simulink model "Benchmark_model"  (R2018a)
settings: Solver=ode1  StartTime=0  StopTime=t_end  FixedStep=simTs  RelTol=1e-3  EnableMultiTasking=on
values from neighbouring files (symbols this model uses):
  driv_rect_time = 0.5    [Initial_parameters.m]
  gamma = 25    [Initial_parameters.m]
  hw_min = 3    [Initial_parameters.m]
  Initial_eng_spd = 0    [Initial_parameters.m]
  Initial_headway = Sensor_FOL_dDist(2)    [Initial_parameters.m]
  Initial_SOC = 50    [Initial_parameters.m]
  Initial_vhcl_spd = 0    [Initial_parameters.m]
  spd_lim = 60    [Initial_parameters.m]
undefined symbols (not defined in the file or in its folder): Route_Distance, Route_Slope
(part 2 of 2)

== matlab function Benchmark_model/Traffic Scenario/V2I information/Data arrangement ==
  data: ego_distance input; State_next1 output; tRemain_next1 output; s2inters_next1 output; State_next2 output; tRemain_next2 output; state_sum input; tRemain_sum input; s2inters_next2 output
function [State_next1,tRemain_next1,s2inters_next1,State_next2,tRemain_next2,s2inters_next2] = fcn(ego_distance,state_sum,tRemain_sum)

%%%% state
TrfLight_TL1_State = state_sum(1);
TrfLight_TL2_State = state_sum(2);
TrfLight_TL3_State = state_sum(3);
TrfLight_TL4_State = state_sum(4);
TrfLight_TL5_State = state_sum(5);
TrfLight_TL6_State = state_sum(6);
TrfLight_TL7_State = state_sum(7);
TrfLight_TL8_State = state_sum(8);
TrfLight_TL9_State = state_sum(9);
TrfLight_TL10_State = state_sum(10);
TrfLight_TL11_State = state_sum(11);
TrfLight_TL12_State = state_sum(12);
TrfLight_TL13_State = state_sum(13);
TrfLight_TL14_State = state_sum(14);
TrfLight_TL15_State = state_sum(15);
TrfLight_TL16_State = state_sum(16);
TrfLight_TL17_State = state_sum(17);
TrfLight_TL18_State = state_sum(18);
TrfLight_TL19_State = state_sum(19);
TrfLight_TL20_State = state_sum(20);
TrfLight_TL21_State = state_sum(21);
TrfLight_TL22_State = state_sum(22);
TrfLight_TL23_State = state_sum(23);
TrfLight_TL24_State = state_sum(24);
TrfLight_TL25_State = state_sum(25);
TrfLight_TL26_State = state_sum(26);

%%%% tRemain
TrfLight_TL1_tRemain = tRemain_sum(1);
TrfLight_TL2_tRemain = tRemain_sum(2);
TrfLight_TL3_tRemain = tRemain_sum(3);
TrfLight_TL4_tRemain = tRemain_sum(4);
TrfLight_TL5_tRemain = tRemain_sum(5);
TrfLight_TL6_tRemain = tRemain_sum(6);
TrfLight_TL7_tRemain = tRemain_sum(7);
TrfLight_TL8_tRemain = tRemain_sum(8);
TrfLight_TL9_tRemain = tRemain_sum(9);
TrfLight_TL10_tRemain = tRemain_sum(10);
TrfLight_TL11_tRemain = tRemain_sum(11);
TrfLight_TL12_tRemain = tRemain_sum(12);
TrfLight_TL13_tRemain = tRemain_sum(13);
TrfLight_TL14_tRemain = tRemain_sum(14);
TrfLight_TL15_tRemain = tRemain_sum(15);
TrfLight_TL16_tRemain = tRemain_sum(16);
TrfLight_TL17_tRemain = tRemain_sum(17);
TrfLight_TL18_tRemain = tRemain_sum(18);
TrfLight_TL19_tRemain = tRemain_sum(19);
TrfLight_TL20_tRemain = tRemain_sum(20);
TrfLight_TL21_tRemain = tRemain_sum(21);
TrfLight_TL22_tRemain = tRemain_sum(22);
TrfLight_TL23_tRemain = tRemain_sum(23);
TrfLight_TL24_tRemain = tRemain_sum(24);
TrfLight_TL25_tRemain = tRemain_sum(25);
TrfLight_TL26_tRemain = tRemain_sum(26);

intersection = [1288;
2358;
2572;
2886;
3066;
3150;
3422;
3784;
4696;
5377;
5576;
6855;
7626;
10162;
10575;
10948;
11201;
11537;
11781;
12302;
12587;
12785;
13032;
13368;
14364;
15082]; % original position of the intersection to the departure


intersection = intersection-3.2; 
% the vehicle length should be considered at the departure 
% and at the departure, the distance of ego vehicle to the first intesection is actually 1284.8 [m]
% so a correction of 3.2 [m] is given.

distination = 16002;


           
if ego_distance < intersection(1)
    TrfLight_State_sum_next1 = TrfLight_TL1_State;
    TrfLight_tRemain_sum_next1 = TrfLight_TL1_tRemain;
    TrfLight_State_sum_next2 = TrfLight_TL2_State;
    TrfLight_tRemain_sum_next2 = TrfLight_TL2_tRemain;  
    ego_vehicle_s2_inters_next1 = intersection(1)-ego_distance;
    ego_vehicle_s2_inters_next2 = intersection(2)-ego_distance;
elseif ego_distance < intersection(2)
    TrfLight_State_sum_next1 = TrfLight_TL2_State;
    TrfLight_tRemain_sum_next1 = TrfLight_TL2_tRemain; 
    TrfLight_State_sum_next2 = TrfLight_TL3_State;
    TrfLight_tRemain_sum_next2 = TrfLight_TL3_tRemain;
    ego_vehicle_s2_inters_next1 = intersection(2)-ego_distance;
    ego_vehicle_s2_inters_next2 = intersection(3)-ego_distance;
elseif ego_distance < intersection(3)
    TrfLight_State_sum_next1 = TrfLight_TL3_State;
    TrfLight_tRemain_sum_next1 = TrfLight_TL3_tRemain; 
    TrfLight_State_sum_next2 = TrfLight_TL4_State;
    TrfLight_tRemain_sum_next2 = TrfLight_TL4_tRemain; 
    ego_vehicle_s2_inters_next1 = intersection(3)-ego_distance;
    ego_vehicle_s2_inters_next2 = intersection(4)-ego_distance;
elseif ego_distance < intersection(4)
    TrfLight_State_sum_next1 = TrfLight_TL4_State;
    TrfLight_tRemain_sum_next1 = TrfLight_TL4_tRemain; 
    TrfLight_State_sum_next2 = TrfLight_TL5_State;
    TrfLight_tRemain_sum_next2 = TrfLight_TL5_tRemain; 
    ego_vehicle_s2_inters_next1 = intersection(4)-ego_distance;
    ego_vehicle_s2_inters_next2 = intersection(5)-ego_distance;
elseif ego_distance < intersection(5)
    TrfLight_State_sum_next1 = TrfLight_TL5_State;
    TrfLight_tRemain_sum_next1 = TrfLight_TL5_tRemain;
    TrfLight_State_sum_next2 = TrfLight_TL6_State;
    TrfLight_tRemain_sum_next2 = TrfLight_TL6_tRemain;
    ego_vehicle_s2_inters_next1 = intersection(5)-ego_distance;
    ego_vehicle_s2_inters_next2 = intersection(6)-ego_distance;
elseif ego_distance < intersection(6)
    TrfLight_State_sum_next1 = TrfLight_TL6_State;
    TrfLight_tRemain_sum_next1 = TrfLight_TL6_tRemain;
    TrfLight_State_sum_next2 = TrfLight_TL7_State;
    TrfLight_tRemain_sum_next2 = TrfLight_TL7_tRemain;
    ego_vehicle_s2_inters_next1 = intersection(6)-ego_distance;
    ego_vehicle_s2_inters_next2 = intersection(7)-ego_distance;
elseif ego_distance < intersection(7)
    TrfLight_State_sum_next1 = TrfLight_TL7_State;
    TrfLight_tRemain_sum_next1 = TrfLight_TL7_tRemain;
    TrfLight_State_sum_next2 = TrfLight_TL8_State;
    TrfLight_tRemain_sum_next2 = TrfLight_TL8_tRemain; 
    ego_vehicle_s2_inters_next1 = intersection(7)-ego_distance;
    ego_vehicle_s2_inters_next2 = intersection(8)-ego_distance;
elseif ego_distance < intersection(8)
    TrfLight_State_sum_next1 = TrfLight_TL8_State;
    TrfLight_tRemain_sum_next1 = TrfLight_TL8_tRemain; 
    TrfLight_State_sum_next2 = TrfLight_TL9_State;
    TrfLight_tRemain_sum_next2 = TrfLight_TL9_tRemain;
    ego_vehicle_s2_inters_next1 = intersection(8)-ego_distance;
    ego_vehicle_s2_inters_next2 = intersection(9)-ego_distance;
elseif ego_distance < intersection(9)
    TrfLight_State_sum_next1 = TrfLight_TL9_State;
    TrfLight_tRemain_sum_next1 = TrfLight_TL9_tRemain; 
    TrfLight_State_sum_next2 = TrfLight_TL10_State;
    TrfLight_tRemain_sum_next2 = TrfLight_TL10_tRemain; 
    ego_vehicle_s2_inters_next1 = intersection(9)-ego_distance;
    ego_vehicle_s2_inters_next2 = intersection(10)-ego_distance;
elseif ego_distance < intersection(10)
    TrfLight_State_sum_next1 = TrfLight_TL10_State;
    TrfLight_tRemain_sum_next1 = TrfLight_TL10_tRemain;
    TrfLight_State_sum_next2 = TrfLight_TL11_State;
    TrfLight_tRemain_sum_next2 = TrfLight_TL11_tRemain; 
    ego_vehicle_s2_inters_next1 = intersection(10)-ego_distance;
    ego_vehicle_s2_inters_next2 = intersection(11)-ego_distance;
elseif ego_distance < intersection(11)
    TrfLight_State_sum_next1 = TrfLight_TL11_State;
    TrfLight_tRemain_sum_next1 = TrfLight_TL11_tRemain; 
    TrfLight_State_sum_next2 = TrfLight_TL12_State;
    TrfLight_tRemain_sum_next2 = TrfLight_TL12_tRemain; 
    ego_vehicle_s2_inters_next1 = intersection(11)-ego_distance;
    ego_vehicle_s2_inters_next2 = intersection(12)-ego_distance;
elseif ego_distance < intersection(12)
    TrfLight_State_sum_next1 = TrfLight_TL12_State;
    TrfLight_tRemain_sum_next1 = TrfLight_TL12_tRemain;
    TrfLight_State_sum_next2 = TrfLight_TL13_State;
    TrfLight_tRemain_sum_next2 = TrfLight_TL13_tRemain;
    ego_vehicle_s2_inters_next1 = intersection(12)-ego_distance;
    ego_vehicle_s2_inters_next2 = intersection(13)-ego_distance;
elseif ego_distance < intersection(13)
    TrfLight_State_sum_next1 = TrfLight_TL13_State;
    TrfLight_tRemain_sum_next1 = TrfLight_TL13_tRemain;
    TrfLight_State_sum_next2 = TrfLight_TL14_State;
    TrfLight_tRemain_sum_next2 = TrfLight_TL14_tRemain;
    ego_vehicle_s2_inters_next1 = intersection(13)-ego_distance;
    ego_vehicle_s2_inters_next2 = intersection(14)-ego_distance;
elseif ego_distance < intersection(14)
    TrfLight_State_sum_next1 = TrfLight_TL14_State;
    TrfLight_tRemain_sum_next1 = TrfLight_TL14_tRemain; 
    TrfLight_State_sum_next2 = TrfLight_TL15_State;
    TrfLight_tRemain_sum_next2 = TrfLight_TL15_tRemain;
    ego_vehicle_s2_inters_next1 = intersection(14)-ego_distance;
    ego_vehicle_s2_inters_next2 = intersection(15)-ego_distance;
elseif ego_distance < intersection(15)
    TrfLight_State_sum_next1 = TrfLight_TL15_State;
    TrfLight_tRemain_sum_next1 = TrfLight_TL15_tRemain; 
    TrfLight_State_sum_next2 = TrfLight_TL16_State;
    TrfLight_tRemain_sum_next2 = TrfLight_TL16_tRemain; 
    ego_vehicle_s2_inters_next1 = intersection(15)-ego_distance;
    ego_vehicle_s2_inters_next2 = intersection(16)-ego_distance;
elseif ego_distance < intersection(16)
    TrfLight_State_sum_next1 = TrfLight_TL16_State;
    TrfLight_tRemain_sum_next1 = TrfLight_TL16_tRemain; 
    TrfLight_State_sum_next2 = TrfLight_TL17_State;
    TrfLight_tRemain_sum_next2 = TrfLight_TL17_tRemain;
    ego_vehicle_s2_inters_next1 = intersection(16)-ego_distance;
    ego_vehicle_s2_inters_next2 = intersection(17)-ego_distance;
elseif ego_distance < intersection(17)
    TrfLight_State_sum_next1 = TrfLight_TL17_State;
    TrfLight_tRemain_sum_next1 = TrfLight_TL17_tRemain; 
    TrfLight_State_sum_next2 = TrfLight_TL18_State;
    TrfLight_tRemain_sum_next2 = TrfLight_TL18_tRemain;
    ego_vehicle_s2_inters_next1 = intersection(17)-ego_distance;
    ego_vehicle_s2_inters_next2 = intersection(18)-ego_distance;
elseif ego_distance < intersection(18)
    TrfLight_State_sum_next1 = TrfLight_TL18_State;
    TrfLight_tRemain_sum_next1 = TrfLight_TL18_tRemain; 
    TrfLight_State_sum_next2 = TrfLight_TL19_State;
    TrfLight_tRemain_sum_next2 = TrfLight_TL19_tRemain;
    ego_vehicle_s2_inters_next1 = intersection(18)-ego_distance;
    ego_vehicle_s2_inters_next2 = intersection(19)-ego_distance;
elseif ego_distance < intersection(19)
    TrfLight_State_sum_next1 = TrfLight_TL19_State;
    TrfLight_tRemain_sum_next1 = TrfLight_TL19_tRemain; 
    TrfLight_State_sum_next2 = TrfLight_TL20_State;
    TrfLight_tRemain_sum_next2 = TrfLight_TL20_tRemain; 
    ego_vehicle_s2_inters_next1 = intersection(19)-ego_distance;
    ego_vehicle_s2_inters_next2 = intersection(20)-ego_distance;
elseif ego_distance < intersection(20)
    TrfLight_State_sum_next1 = TrfLight_TL20_State;
    TrfLight_tRemain_sum_next1 = TrfLight_TL20_tRemain; 
    TrfLight_State_sum_next2 = TrfLight_TL21_State;
    TrfLight_tRemain_sum_next2 = TrfLight_TL21_tRemain; 
    ego_vehicle_s2_inters_next1 = intersection(20)-ego_distance;
    ego_vehicle_s2_inters_next2 = intersection(21)-ego_distance;
elseif ego_distance < intersection(21)
    TrfLight_State_sum_next1 = TrfLight_TL21_State;
    TrfLight_tRemain_sum_next1 = TrfLight_TL21_tRemain;
    TrfLight_State_sum_next2 = TrfLight_TL22_State;
    TrfLight_tRemain_sum_next2 = TrfLight_TL22_tRemain;
    ego_vehicle_s2_inters_next1 = intersection(21)-ego_distance;
    ego_vehicle_s2_inters_next2 = intersection(22)-ego_distance;
elseif ego_distance < intersection(22)
    TrfLight_State_sum_next1 = TrfLight_TL22_State;
    TrfLight_tRemain_sum_next1 = TrfLight_TL22_tRemain; 
    TrfLight_State_sum_next2 = TrfLight_TL23_State;
    TrfLight_tRemain_sum_next2 = TrfLight_TL23_tRemain;
    ego_vehicle_s2_inters_next1 = intersection(22)-ego_distance;
    ego_vehicle_s2_inters_next2 = intersection(23)-ego_distance;
elseif ego_distance < intersection(23)
    TrfLight_State_sum_next1 = TrfLight_TL23_State;
    TrfLight_tRemain_sum_next1 = TrfLight_TL23_tRemain; 
    TrfLight_State_sum_next2 = TrfLight_TL24_State;
    TrfLight_tRemain_sum_next2 = TrfLight_TL24_tRemain;
    ego_vehicle_s2_inters_next1 = intersection(23)-ego_distance;
    ego_vehicle_s2_inters_next2 = intersection(24)-ego_distance;
elseif ego_distance < intersection(24)
    TrfLight_State_sum_next1 = TrfLight_TL24_State;
    TrfLight_tRemain_sum_next1 = TrfLight_TL24_tRemain; 
    TrfLight_State_sum_next2 = TrfLight_TL25_State;
    TrfLight_tRemain_sum_next2 = TrfLight_TL25_tRemain;
    ego_vehicle_s2_inters_next1 = intersection(24)-ego_distance;
    ego_vehicle_s2_inters_next2 = intersection(25)-ego_distance;
elseif ego_distance < intersection(25)
    TrfLight_State_sum_next1 = TrfLight_TL25_State;
    TrfLight_tRemain_sum_next1 = TrfLight_TL25_tRemain; 
    TrfLight_State_sum_next2 = TrfLight_TL26_State;
    TrfLight_tRemain_sum_next2 = TrfLight_TL26_tRemain;
    ego_vehicle_s2_inters_next1 = intersection(25)-ego_distance;
    ego_vehicle_s2_inters_next2 = intersection(26)-ego_distance;
elseif ego_distance < intersection(26)
    TrfLight_State_sum_next1 = TrfLight_TL26_State;
    TrfLight_tRemain_sum_next1 = TrfLight_TL26_tRemain; 
    TrfLight_State_sum_next2 = nan;
    TrfLight_tRemain_sum_next2 = nan;
    ego_vehicle_s2_inters_next1 = intersection(26)-ego_distance;
    ego_vehicle_s2_inters_next2 = distination-ego_distance;
else
    TrfLight_State_sum_next1 = nan;
    TrfLight_tRemain_sum_next1 = nan; 
    TrfLight_State_sum_next2 = nan;
    TrfLight_tRemain_sum_next2 = nan;
    ego_vehicle_s2_inters_next1 = distination-ego_distance;
    ego_vehicle_s2_inters_next2 = nan;
end

State_next1 = TrfLight_State_sum_next1;
tRemain_next1 = TrfLight_tRemain_sum_next1;
s2inters_next1 = ego_vehicle_s2_inters_next1;

State_next2 = TrfLight_State_sum_next2;
tRemain_next2 = TrfLight_tRemain_sum_next2;
s2inters_next2 = ego_vehicle_s2_inters_next2;

== matlab function Benchmark_model/Controller(Sample)/MATLAB Function ==
  data: V2X input; Te_act output; Tg_act output; Tm_act output; Fb_act output; Vvel_s input; Ne_ini input; Vvel_ini input; SOC_constraint output; SOC_ini input
function [Te_act,Tg_act,Tm_act,Fb_act,SOC_constraint] = Upper_controller(V2X,Vvel_s,Ne_ini,Vvel_ini,SOC_ini)
% load('DATA/HEV_powertrain_parameters.mat');%混合动力参数
% load('DATA/Route_slope_parameters.mat');%道路坡度信息
%--------------------------------------------------------------------------
coder.extrinsic('evalin');
Route_Distence=evalin('base','Route_Distence');
Route_Slope=evalin('base','Route_Slope');
MG2_MaxMintorque_Spd=evalin('base','MG2_MaxMintorque_Spd');
MG2_MaxMintorque_MaxTrq=evalin('base','MG2_MaxMintorque_MaxTrq');
MG2_MaxMintorque_MinTrq=evalin('base','MG2_MaxMintorque_MinTrq');
Maxtorque_EngSpd=evalin('base','Maxtorque_EngSpd');
Maxtorque_EngTrq=evalin('base','Maxtorque_EngTrq');
MG1_MaxMintorque_Spd=evalin('base','MG1_MaxMintorque_Spd');
MG1_MaxMintorque_MaxTrq=evalin('base','MG1_MaxMintorque_MaxTrq');
MG1_MaxMintorque_MinTrq=evalin('base','MG1_MaxMintorque_MinTrq');                             
MG1_MechanicalLoss_Spd=evalin('base','MG1_MechanicalLoss_Spd');
MG1_MechanicalLoss_Trq=evalin('base','MG1_MechanicalLoss_Trq');
MG1_MechanicalLoss_Marix=evalin('base','MG1_MechanicalLoss_Marix');
MG2_MechanicalLoss_Spd=evalin('base','MG2_MechanicalLoss_Spd');
MG2_MechanicalLoss_Trq=evalin('base','MG2_MechanicalLoss_Trq');
MG2_MechanicalLoss_Marix=evalin('base','MG2_MechanicalLoss_Marix');          
FuelConsmp_EngSpd=evalin('base','FuelConsmp_EngSpd');
FuelConsmp_EngTrq=evalin('base','FuelConsmp_EngTrq');
FuelConsmp_Rate_Matrix=evalin('base','FuelConsmp_Rate_Matrix');
% =evalin('base','');
% =evalin('base','');
% =evalin('base','');
%% 基本参数
N_p_s=20;%下层预测步数
%----------------------------电池特性参数----------------------------------
Paux=0.2793*10^3;%辅助设备功率 Unit:[W]
Bat.C=23.275*3600;%电池电量 Unit:[A*s]
% 开环电压参数 [V]
%V_oc=(x<=.12)*(a1*x+b1)+(.12<x & x<=.21)*(a2*x+b2)+...
% (.21<x & x<=.25)*(a3*x+b3)+(.25<x & x<=.30)*(a4*x+b4)+...
% (.30<x & x<=.40)*(a5*x+b5)+(.40<x & x<=.50)*(a6*x+b6)+...
% (.50<x & x<=.56)*(a7*x+b7)+(.56<x & x<=.72)*(a8*x+b8)+...
% (.72<x)*(a9*x+b9);
Bat.V.a1 =      0.5472;
Bat.V.a2 =      0.8964;
Bat.V.a3 =      0.6156;
Bat.V.a4 =      0.4039;
Bat.V.a5 =      0.3432;
Bat.V.a6 =      0.5366;
Bat.V.a7 =       1.097;
Bat.V.a8 =       1.024;
Bat.V.a9 =       1.219;
Bat.V.b1 =       325.4;
Bat.V.b2 =         321;
Bat.V.b3 =       326.9;
Bat.V.b4 =       332.2;
Bat.V.b5 =       333.9;
Bat.V.b6 =         326;
Bat.V.b7 =       298.2;
Bat.V.b8 =       302.1;
Bat.V.b9 =         288;
% 内阻参数 [\ohm]
% R_int=(x<=.12)*(a1*x+b1)+(.12<x & x<=.18)*(a2*x+b2)+...
%     (.18<x & x<=25)*(a3*x+b3)+(.25<x & x<=.29)*(a4*x+b4)+...
%     (.29<x & x<=.37)*(a5*x+b5)+(.37<x & x<=.54)*(a6*x+b6)+...
%     (.54<x & x<=.71)*(a7*x+b7)+(.71<x)*(a8*x+b8);
Bat.R.a1 =   -0.001596;
Bat.R.a2 =   -0.001118;
Bat.R.a3 =   -0.000912;
Bat.R.a4 =   -0.000684;
Bat.R.a5 =  -0.0002286;
Bat.R.a6 =  -0.0004554;
Bat.R.a7 =   -0.000228;
Bat.R.a8 =  -5.197e-19;
Bat.R.b1 =      0.1995;
Bat.R.b2 =      0.1935;
Bat.R.b3 =        0.19;
Bat.R.b4 =      0.1843;
Bat.R.b5 =       0.171;
Bat.R.b6 =      0.1795;
Bat.R.b7 =      0.1672;
Bat.R.b8 =       0.151;
% ---------------------------传动系统参数---------------------------%
%Unit:[kgm^2]
I.e=0.1420;%Inertia of engine
I.c=0;%Inertia of carrier（这里没给，我认为pdf里Ie就是这里Ie+I.c）
I.g=0.0154;%Inertia of MG1 and sun
I.m=0.0074;%Inertia of MG2 and reduction
I.t=3.12;%Inertia of tire and drive-shift
%Unit:[kg]
M=1700;%汽车总质量
%Unit:[m/s^2]
g=9.81;
%Unit:[m]
R.f1=19e-3;
R.f2=75e-3;
R.c1=65e-3;
R.c2=53e-3;
R.s=30e-3;
R.r=78e-3;
R.m=17e-3;
R.t=317.25e-3;%轮胎半径（pdf文件这里错了）
Rc12t=R.c1*R.f1/R.c2/R.f2;%齿圈到车轮传动关系
kph2mps=1/3.6;%km/h->m/s换算关系
rpm2rads=pi/30;%rpm->rad/s 换算关系
simTs=0.01;%采样时间
g=9.807;%重力加速度
%% ---------------------转速传动关系（行星齿轮）-------------------- %
%W2T*[omega_g;omega_e;omega_r;F]=[-Tg;Te;Tm*R.c2*R.f2/R.m/R.f1-Fb-Tload;0];
% omega_e与omega_r
W2T=[I.g 0 0 -R.s;
    0 I.c+I.e 0 (R.s+R.r);
    0 0 R.c1*R.f1/R.c2/R.f2*(M*R.t^2+I.t)+R.c1*R.c2*R.f2/R.m^2/R.f1*I.m -R.r*R.c2*R.f2/R.c1/R.f1;
    R.s -(R.s+R.r) R.r 0];%omega2torque
T2W=inv(W2T);%torque2omega

% A=eye(2);%状态转移矩阵
% Bu=[-T2W(2,1) T2W(2,2) R.c2*R.f2/R.m/R.f1*T2W(2,3) -T2W(2,3);
%     -T2W(3,1) T2W(3,2) R.c2*R.f2/R.m/R.f1*T2W(3,3) -T2W(3,3)];
% Bw=[-T2W(2,3);
%     -T2W(3,3)];
%% ---------------------------控制器设计---------------------------- %
%三阶动态方程（soc、omega_e,omega_r）
%控制量：Tg、Te、Tm、Fb；状态量：soc、omega_e,omega_r
Cr=0.006434;%摩擦系数
beta=0.0291;%风阻系数
%T_load=Mgsin(theta)*R.t+Mgcos(theta)*Cr*R.t+beta*v_vel^2
%% V_vel_s：本车预测车速 SOC：当前电池SOC值
SOC_final=0.5;%预测终端SOC期望值
SOC_tol=1e-2;%终端SOC允许最大偏差
N_p=length(Vvel_s);%预测步数
Nr_ref=Vvel_s*kph2mps/R.t/Rc12t;%预测时域内齿圈转速期望值
%当前状态量值
SOC=SOC_ini/100;%电池SOC[-]
Ne=Ne_ini;%发动机转速[rpm]
Nr_ini=Vvel_ini*kph2mps/R.t/Rc12t;%当前齿圈转速[ini均为当前值]
d_ini=V2X(2);%b本车当前位置
theta_ini=interp1(Route_Distence,Route_Slope,d_ini);%当前位置道路坡度
% Nr_ref=[Nr_ini,Nr_ref];%齿圈转速期望值加入当前转速，方便之后计算
%-------------------------------------------------------------------------%
%用于预测时域内循环
theta=theta_ini;%当前道路倾角
d=d_ini;%驾驶行程
% omega=[omega_e;omega_r];
Num_MG2=100;%电机2扭力分100点
Num_Eng=100;%发动机扭力分100个点
%% PMP 相关量定义
lambda_max=50;
lambda_min=-lambda_max;
lambda=lambda_min;%协态变量
Max_iter=50;%最大迭代次数
%% lambda 下界情况SOC终端情况
lambda=lambda_min;
% 预测计算
for i=1:N_p-1
    %电池相关物理量
    V_oc=(SOC<=.12)*(Bat.V.a1*SOC+Bat.V.b1)+(.12<SOC & SOC<=.21)*(Bat.V.a2*SOC+Bat.V.b2)+...
        (.21<SOC & SOC<=.25)*(Bat.V.a3*SOC+Bat.V.b3)+(.25<SOC & SOC<=.30)*(Bat.V.a4*SOC+Bat.V.b4)+...
        (.30<SOC & SOC<=.40)*(Bat.V.a5*SOC+Bat.V.b5)+(.40<SOC & SOC<=.50)*(Bat.V.a6*SOC+Bat.V.b6)+...
        (.50<SOC & SOC<=.56)*(Bat.V.a7*SOC+Bat.V.b7)+(.56<SOC & SOC<=.72)*(Bat.V.a8*SOC+Bat.V.b8)+...
        (.72<SOC)*(Bat.V.a9*SOC+Bat.V.b9);%当前电池开路电压
    R_int=(SOC<=.12)*(Bat.R.a1*SOC+Bat.R.b1)+(.12<SOC & SOC<=.18)*(Bat.R.a2*SOC+Bat.R.b2)+...
        (.18<SOC & SOC<=.25)*(Bat.R.a3*SOC+Bat.R.b3)+(.25<SOC & SOC<=.29)*(Bat.R.a4*SOC+Bat.R.b4)+...
        (.29<SOC & SOC<=.37)*(Bat.R.a5*SOC+Bat.R.b5)+(.37<SOC & SOC<=.54)*(Bat.R.a6*SOC+Bat.R.b6)+...
        (.54<SOC & SOC<=.71)*(Bat.R.a7*SOC+Bat.R.b7)+(.71<SOC)*(Bat.R.a8*SOC+Bat.R.b8);%当前电池内阻
    %齿圈相关物理量
    Nr_vol=Nr_ref(i);%预测i-1时刻齿圈速度
    Nr_acc=(Nr_ref(i+1)-Nr_ref(i))/simTs;%预测i-1时刻齿圈加速度
    %电机2（整车）相关物理量
    Tm_max=interp1(MG2_MaxMintorque_Spd,MG2_MaxMintorque_MaxTrq,Nr_vol*R.c1/R.m/rpm2rads);%电机2当前转速最大扭力[+]
    Tm_min=interp1(MG2_MaxMintorque_Spd,MG2_MaxMintorque_MinTrq,Nr_vol*R.c1/R.m/rpm2rads);%电机2当前转速最大扭力[-]
    Tm_grid=linspace(Tm_min,Tm_max,Num_MG2);
    T_load=M*g*sin(theta)*R.t+M*g*cos(theta)*Cr*R.t+...
        beta*(Nr_vol*R.c1*R.f1*R.t/R.c2/R.f2)^2;
    %发动机相关物理量
    Te_max=interp1(Maxtorque_EngSpd,Maxtorque_EngTrq,Ne/rpm2rads);%发动机当前转速最大扭力
    Te_grid=linspace(0,Te_max,Num_Eng);
    %电机1相关物理量
    Ng_act=((R.s+R.r)*Ne-R.r*Nr_vol)/R.s;%预测第i-1步实际转速
    if Ng_act<0
        Ng_vir=-Ng_act;
    else
        Ng_vir=Ng_act;
    end
    Tg_max=interp1(MG1_MaxMintorque_Spd,MG1_MaxMintorque_MaxTrq,Ng_vir/rpm2rads);%电机1当前转速最大扭力[+]
    Tg_min=interp1(MG1_MaxMintorque_Spd,MG1_MaxMintorque_MinTrq,Ng_vir/rpm2rads);%电机1当前转速最大扭力[-]
    for j=1:length(Tm_grid)%循环电机2可能的所有扭矩
        Tm=Tm_grid(j);
        for k=1:length(Te_grid)%循环发动机可能的所有扭矩
            Te=Te_grid(k);
            if Te>0
                Fb=0;
                Fb_Matrix(j,k)=0;
                Tg=(T2W(3,2)*Te+R.c2*R.f2/R.m/R.f1*T2W(3,3)*Tm-...
                    T2W(3,3)*Fb-T2W(3,3)*T_load-Nr_acc)/T2W(3,1);
                if (Tg>=Tg_min && Tg<=Tg_max)
                    Tg_Matrix(j,k)=Tg;
                else
                    Tg_Matrix(j,k)=nan;
                end
            else
                Fb_ass=0;
                Tg_ass=(T2W(3,2)*Te+R.c2*R.f2/R.m/R.f1*T2W(3,3)*Tm-...
                    T2W(3,3)*Fb_ass-T2W(3,3)*T_load-Nr_acc)/T2W(3,1);
                if (Tg_ass>=Tg_min && Tg_ass<=Tg_max)     %制动能量全部回收
                    Tg_Matrix(j,k)=Tg_ass;
                    Fb_Matrix(j,k)=Fb_ass;
                elseif Tg_ass>=Tg_max           %刹车系统承担一部分制动效果
                    Tg_Matrix(j,k)=Tg_max;
                    Fb_Matrix(j,k)=(T2W(3,2)*Te+R.c2*R.f2/R.m/R.f1*T2W(3,3)*Tm-...
                    T2W(3,3)*T_load-Nr_acc-T2W(3,1)*Tg_max)/T2W(3,3);
                else
%                     disp('Error！');
                    Tg_Matrix(j,k)=nan;
                    Fb_Matrix(j,k)=nan;
                end
            end
            if isnan(Tg_Matrix(j,k))
                H(j,k)=nan;
            else
                MG1_heat_loss=interp2(MG1_MechanicalLoss_Spd,MG1_MechanicalLoss_Trq,...
                    MG1_MechanicalLoss_Marix,Ng_vir/rpm2rads,Tg);%电机1热损失
                MG2_heat_loss=interp2(MG2_MechanicalLoss_Spd,MG2_MechanicalLoss_Trq,...
                    MG2_MechanicalLoss_Marix,Nr_vol*R.c1/R.m/rpm2rads,Tm);%电机2热损失
                MG1_Mech_power=Ng_vir*Tg;%单位W
                MG2_Mech_power=Nr_vol*R.c1/R.m*Tm;%单位W
                P_bat_MG1=MG1_Mech_power+MG1_heat_loss;%电机1发/耗电量
                P_bat_MG2=MG2_Mech_power+MG2_heat_loss;%电机2发/耗电量
                P_bat=P_bat_MG1+P_bat_MG2+Paux;%电池总供电量
                H(j,k)=interp2(FuelConsmp_EngSpd,FuelConsmp_EngTrq,...
                    FuelConsmp_Rate_Matrix,Ne,Te)+lambda*(-(V_oc-(V_oc^2-4*P_bat*...
                    R_int)^0.5)/(2*Bat.C*R_int))+5/(1+exp(1000*SOC-90))+...
                    5/(1+exp(910-1000*SOC));%协态方程+状态量软约束
            end
        end%发动机扭矩循环结束
    end%电机2扭矩循环结束
    [value1,ind1]=min(H,[],1);%对哈密顿按列取极小值[ind1:行]
    [value2,ind2]=min(value1);%求得最优的哈密顿值对应的控制量序列[ind2:列]
    %最优控制量给入
    Te_opt=Te_grid(ind2);%对应的发动机最佳扭矩
    Tm_opt=Tm_opt(ind(ind2));%对应的电机2最佳扭矩
    Tg_opt=Tg_Matrix(ind(ind2),ind2);%对应的电机1最佳扭矩
    Fb_opt=Fb_Matrix(ind(ind2),ind2);%对应的最佳制动力
    %供电最优分配
    MG1_heat_loss_opt=interp2(MG1_MechanicalLoss_Spd,MG1_MechanicalLoss_Trq,...
        MG1_MechanicalLoss_Marix,Ng_vir/rpm2rads,Tg_opt);%电机1热损失
    MG2_heat_loss_opt=interp2(MG2_MechanicalLoss_Spd,MG2_MechanicalLoss_Trq,...
        MG2_MechanicalLoss_Marix,Nr_vol*R.c1/R.m/rpm2rads,Tm_opt);%电机2热损失
    MG1_Mech_power_opt=Ng_vir*Tg_opt;%单位W
    MG2_Mech_power_opt=Nr_vol*R.c1/R.m*Tm_opt;%单位W
    P_bat_MG1_opt=MG1_Mech_power_opt+MG1_heat_loss_opt;%电机1发/耗电量
    P_bat_MG2_opt=MG2_Mech_power_opt+MG2_heat_loss_opt;%电机2发/耗电量
    P_bat_opt=P_bat_MG1_opt+P_bat_MG2_opt+Paux;%电池总供电量
    %状态量的更新【第i步预测量值】
    %协态更新
    dot_V_oc=(SOC<=.12)*Bat.V.a1+(.12<SOC & SOC<=.21)*Bat.V.a2+...
        (.21<SOC & SOC<=.25)*Bat.V.a3+(.25<SOC & SOC<=.30)*Bat.V.a4*SOC+...
        (.30<SOC & SOC<=.40)*Bat.V.a5+(.40<SOC & SOC<=.50)*Bat.V.a6+...
        (.50<SOC & SOC<=.56)*Bat.V.a7+(.56<SOC & SOC<=.72)*Bat.V.a8+...
        (.72<SOC)*Bat.V.a9;%开路电压对SOC求导
    dot_R_int=(SOC<=.12)*Bat.R.a1+(.12<SOC & SOC<=.18)*Bat.R.a2+...
        (.18<SOC & SOC<=.25)*Bat.R.a3+(.25<SOC & SOC<=.29)*Bat.R.a4+...
        (.29<SOC & SOC<=.37)*Bat.R.a5+(.37<SOC & SOC<=.54)*Bat.R.a6+...
        (.54<SOC & SOC<=.71)*Bat.R.a7+(.71<SOC)*Bat.R.a8;%内阻对SOC求导
    if (1+exp(910-1000*SOC))^2==inf
        item=0;
    else
        item=5000*exp(1000*SOC-90)/(1+exp(1000*SOC-90))^2-...
            5000*exp(910-1000*SOC)/(1+exp(910-1000*SOC))^2;%状态约束项偏导
    end
    dot_lambda=item+lambda*(((dot_V_oc-0.5*(V_oc^2-4*P_bat_opt*R_int)^(-0.5)*...
        (2*V_oc*dot_V_oc-4*P_bat_opt*dot_R_int))*2*Bat.C*R_int)-...
        (V_oc-(V_oc^2-4*P_bat_opt*R_int)^0.5)*2*Bat.C*dot_R_int)/...
        (2*Bat.C*R_int)^2;%协态方程
    lambda=lambda+dot_lambda*simTs;
    %SOC
    SOC=SOC+(-(V_oc-(V_oc^2-4*P_bat_opt*R_int)^0.5)/(2*Bat.C*R_int))*simTs;
    %Ne
    Ne=Ne+(-T2W(2,1)*Tg_opt+T2W(2,2)*Te_opt+R.c2*R.f2/R.m/R.f1*T2W(2,3)*Tm_opt-...
        T2W(2,3)*Fb_opt-T2W(2,3)*T_load)*simTs;
    %其他量更新
    %车辆当前位置
    d=d+(Nr_ref(i)+Nr_ref(i+1))/2*(R.c1*R.f1*R.t/R.c2/R.f2)*simTs;
    %道路倾角
    theta=interp1(Route_Distence,Route_Slope,d);
end%预测循环结束
SOC_end_Lb=SOC;%下界lambda对应终端SOC
if abs(SOC_end_Lb-SOC_final)<=SOC_tol
    lambda_opt=lambda_min;
    flag=0;
else
    flag=1;
end
while flag
    for iter=0:Max_iter
        lambda_ini=(lambda_min+lambda_max)/2;
        lambda=lambda_ini;
        % 预测计算
        for i=1:N_p-1
            %电池相关物理量
            V_oc=(SOC<=.12)*(Bat.V.a1*SOC+Bat.V.b1)+(.12<SOC & SOC<=.21)*(Bat.V.a2*SOC+Bat.V.b2)+...
                (.21<SOC & SOC<=.25)*(Bat.V.a3*SOC+Bat.V.b3)+(.25<SOC & SOC<=.30)*(Bat.V.a4*SOC+Bat.V.b4)+...
                (.30<SOC & SOC<=.40)*(Bat.V.a5*SOC+Bat.V.b5)+(.40<SOC & SOC<=.50)*(Bat.V.a6*SOC+Bat.V.b6)+...
                (.50<SOC & SOC<=.56)*(Bat.V.a7*SOC+Bat.V.b7)+(.56<SOC & SOC<=.72)*(Bat.V.a8*SOC+Bat.V.b8)+...
                (.72<SOC)*(Bat.V.a9*SOC+Bat.V.b9);%当前电池开路电压
            R_int=(SOC<=.12)*(Bat.R.a1*SOC+Bat.R.b1)+(.12<SOC & SOC<=.18)*(Bat.R.a2*SOC+Bat.R.b2)+...
                (.18<SOC & SOC<=.25)*(Bat.R.a3*SOC+Bat.R.b3)+(.25<SOC & SOC<=.29)*(Bat.R.a4*SOC+Bat.R.b4)+...
                (.29<SOC & SOC<=.37)*(Bat.R.a5*SOC+Bat.R.b5)+(.37<SOC & SOC<=.54)*(Bat.R.a6*SOC+Bat.R.b6)+...
                (.54<SOC & SOC<=.71)*(Bat.R.a7*SOC+Bat.R.b7)+(.71<SOC)*(Bat.R.a8*SOC+Bat.R.b8);%当前电池内阻
            %齿圈相关物理量
            Nr_vol=Nr_ref(i);%预测i-1时刻齿圈速度
            Nr_acc=(Nr_ref(i+1)-Nr_ref(i))/simTs;%预测i-1时刻齿圈加速度
            %电机2（整车）相关物理量
            Tm_max=interp1(MG2_MaxMintorque_Spd,MG2_MaxMintorque_MaxTrq,Nr_vol*R.c1/R.m/rpm2rads);%电机2当前转速最大扭力[+]
            Tm_min=interp1(MG2_MaxMintorque_Spd,MG2_MaxMintorque_MinTrq,Nr_vol*R.c1/R.m/rpm2rads);%电机2当前转速最大扭力[-]
            Tm_grid=linspace(Tm_min,Tm_max,Num_MG2);
            T_load=M*g*sin(theta)*R.t+M*g*cos(theta)*Cr*R.t+...
                beta*(Nr_vol*R.c1*R.f1*R.t/R.c2/R.f2)^2;
            %发动机相关物理量
            Te_max=interp1(Maxtorque_EngSpd,Maxtorque_EngTrq,Ne/rpm2rads);%发动机当前转速最大扭力
            Te_grid=linspace(0,Te_max,Num_Eng);
            %电机1相关物理量
            Ng_act=((R.s+R.r)*Ne-R.r*Nr_vol)/R.s;%预测第i-1步实际转速
            if Ng_act<0
                Ng_vir=-Ng_act;
            else
                Ng_vir=Ng_act;
            end
            Tg_max=interp1(MG1_MaxMintorque_Spd,MG1_MaxMintorque_MaxTrq,Ng_vir/rpm2rads);%电机1当前转速最大扭力[+]
            Tg_min=interp1(MG1_MaxMintorque_Spd,MG1_MaxMintorque_MinTrq,Ng_vir/rpm2rads);%电机1当前转速最大扭力[-]
            for j=1:length(Tm_grid)%循环电机2可能的所有扭矩
                Tm=Tm_grid(j);
                for k=1:length(Te_grid)%循环发动机可能的所有扭矩
                    Te=Te_grid(k);
                    if Te>0
                        Fb=0;
                        Fb_Matrix(j,k)=0;
                        Tg=(T2W(3,2)*Te+R.c2*R.f2/R.m/R.f1*T2W(3,3)*Tm-...
                            T2W(3,3)*Fb-T2W(3,3)*T_load-Nr_acc)/T2W(3,1);
                        if (Tg>=Tg_min && Tg<=Tg_max)
                            Tg_Matrix(j,k)=Tg;
                        else
                            Tg_Matrix(j,k)=nan;
                        end
                    else
                        Fb_ass=0;
                        Tg_ass=(T2W(3,2)*Te+R.c2*R.f2/R.m/R.f1*T2W(3,3)*Tm-...
                            T2W(3,3)*Fb_ass-T2W(3,3)*T_load-Nr_acc)/T2W(3,1);
                        if (Tg_ass>=Tg_min && Tg_ass<=Tg_max)     %制动能量全部回收
                            Tg_Matrix(j,k)=Tg_ass;
                            Fb_Matrix(j,k)=Fb_ass;
                        elseif Tg_ass>=Tg_max           %刹车系统承担一部分制动效果
                            Tg_Matrix(j,k)=Tg_max;
                            Fb_Matrix(j,k)=(T2W(3,2)*Te+R.c2*R.f2/R.m/R.f1*T2W(3,3)*Tm-...
                                T2W(3,3)*T_load-Nr_acc-T2W(3,1)*Tg_max)/T2W(3,3);
                        else
%                             disp('Error！');
                            Tg_Matrix(j,k)=nan;
                            Fb_Matrix(j,k)=nan;
                        end
                    end
                    if isnan(Tg_Matrix(j,k))
                        H(j,k)=nan;
                    else
                        MG1_heat_loss=interp2(MG1_MechanicalLoss_Spd,MG1_MechanicalLoss_Trq,...
                            MG1_MechanicalLoss_Marix,Ng_vir/rpm2rads,Tg);%电机1热损失
                        MG2_heat_loss=interp2(MG2_MechanicalLoss_Spd,MG2_MechanicalLoss_Trq,...
                            MG2_MechanicalLoss_Marix,Nr_vol*R.c1/R.m/rpm2rads,Tm);%电机2热损失
                        MG1_Mech_power=Ng_vir*Tg;%单位W
                        MG2_Mech_power=Nr_vol*R.c1/R.m*Tm;%单位W
                        P_bat_MG1=MG1_Mech_power+MG1_heat_loss;%电机1发/耗电量
                        P_bat_MG2=MG2_Mech_power+MG2_heat_loss;%电机2发/耗电量
                        P_bat=P_bat_MG1+P_bat_MG2+Paux;%电池总供电量
                        H(j,k)=interp2(FuelConsmp_EngSpd,FuelConsmp_EngTrq,...
                            FuelConsmp_Rate_Matrix,Ne,Te)+lambda*(-(V_oc-(V_oc^2-4*P_bat*...
                            R_int)^0.5)/(2*Bat.C*R_int))+5/(1+exp(1000*SOC-90))+...
                            5/(1+exp(910-1000*SOC));%协态方程+状态量软约束
                    end
                end%发动机扭矩循环结束
            end%电机2扭矩循环结束
            [value1,ind1]=min(H,[],1);%对哈密顿按列取极小值[ind1:行]
            [value2,ind2]=min(value1);%求得最优的哈密顿值对应的控制量序列[ind2:列]
            %最优控制量给入
            Te_opt=Te_grid(ind2);%对应的发动机最佳扭矩
            Tm_opt=Tm_opt(ind(ind2));%对应的电机2最佳扭矩
            Tg_opt=Tg_Matrix(ind(ind2),ind2);%对应的电机1最佳扭矩
            Fb_opt=Fb_Matrix(ind(ind2),ind2);%对应的最佳制动力
            %供电最优分配
            MG1_heat_loss_opt=interp2(MG1_MechanicalLoss_Spd,MG1_MechanicalLoss_Trq,...
                MG1_MechanicalLoss_Marix,Ng_vir/rpm2rads,Tg_opt);%电机1热损失
            MG2_heat_loss_opt=interp2(MG2_MechanicalLoss_Spd,MG2_MechanicalLoss_Trq,...
                MG2_MechanicalLoss_Marix,Nr_vol*R.c1/R.m/rpm2rads,Tm_opt);%电机2热损失
            MG1_Mech_power_opt=Ng_vir*Tg_opt;%单位W
            MG2_Mech_power_opt=Nr_vol*R.c1/R.m*Tm_opt;%单位W
            P_bat_MG1_opt=MG1_Mech_power_opt+MG1_heat_loss_opt;%电机1发/耗电量
            P_bat_MG2_opt=MG2_Mech_power_opt+MG2_heat_loss_opt;%电机2发/耗电量
            P_bat_opt=P_bat_MG1_opt+P_bat_MG2_opt+Paux;%电池总供电量
            %状态量的更新【第i步预测量值】
            %协态更新
            dot_V_oc=(SOC<=.12)*Bat.V.a1+(.12<SOC & SOC<=.21)*Bat.V.a2+...
                (.21<SOC & SOC<=.25)*Bat.V.a3+(.25<SOC & SOC<=.30)*Bat.V.a4*SOC+...
                (.30<SOC & SOC<=.40)*Bat.V.a5+(.40<SOC & SOC<=.50)*Bat.V.a6+...
                (.50<SOC & SOC<=.56)*Bat.V.a7+(.56<SOC & SOC<=.72)*Bat.V.a8+...
                (.72<SOC)*Bat.V.a9;%开路电压对SOC求导
            dot_R_int=(SOC<=.12)*Bat.R.a1+(.12<SOC & SOC<=.18)*Bat.R.a2+...
                (.18<SOC & SOC<=.25)*Bat.R.a3+(.25<SOC & SOC<=.29)*Bat.R.a4+...
                (.29<SOC & SOC<=.37)*Bat.R.a5+(.37<SOC & SOC<=.54)*Bat.R.a6+...
                (.54<SOC & SOC<=.71)*Bat.R.a7+(.71<SOC)*Bat.R.a8;%内阻对SOC求导
            if (1+exp(910-1000*SOC))^2==inf
                item=0;
            else
                item=5000*exp(1000*SOC-90)/(1+exp(1000*SOC-90))^2-...
                    5000*exp(910-1000*SOC)/(1+exp(910-1000*SOC))^2;%状态约束项偏导
            end
            dot_lambda=item+lambda*(((dot_V_oc-0.5*(V_oc^2-4*P_bat_opt*R_int)^(-0.5)*...
                (2*V_oc*dot_V_oc-4*P_bat_opt*dot_R_int))*2*Bat.C*R_int)-...
                (V_oc-(V_oc^2-4*P_bat_opt*R_int)^0.5)*2*Bat.C*dot_R_int)/...
                (2*Bat.C*R_int)^2;%协态方程
            lambda=lambda+dot_lambda*simTs;
            %SOC
            SOC=SOC+(-(V_oc-(V_oc^2-4*P_bat_opt*R_int)^0.5)/(2*Bat.C*R_int))*simTs;
            %Ne
            Ne=Ne+(-T2W(2,1)*Tg_opt+T2W(2,2)*Te_opt+R.c2*R.f2/R.m/R.f1*T2W(2,3)*Tm_opt-...
                T2W(2,3)*Fb_opt-T2W(2,3)*T_load)*simTs;
            %其他量更新
            %车辆当前位置
            d=d+(Nr_ref(i)+Nr_ref(i+1))/2*(R.c1*R.f1*R.t/R.c2/R.f2)*simTs;
            %道路倾角
            theta=interp1(Route_Distence,Route_Slope,d);
        end%预测循环结束
        SOC_end=SOC;
        if abs(SOC_end-SOC_final)<=SOC_final%在SOC容许范围内 打靶结束
            lambda_opt=lambda_ini;
            flag=0;
            break;
        elseif (SOC_end_Lb-SOC_final)*(SOC_end-SOC_final)<0%在SOC容许范围外，二分打靶
            lambda_max=lambda_ini;
        elseif (SOC_end_Lb-SOC_final)*(SOC_end-SOC_final)>0
            lambda_min=lambda_ini;
            SOC_end_Lb=SOC_end;
        end
    end%打靶循环结束
    if iter==Max_iter
        lambda_opt=lambda_ini;
        flag=0;
    end
end%判断是否退出while循环符
lambda=lambda_opt;%打靶法求得初值
for i=1:N_p_s
    %电池相关物理量
    V_oc=(SOC<=.12)*(Bat.V.a1*SOC+Bat.V.b1)+(.12<SOC & SOC<=.21)*(Bat.V.a2*SOC+Bat.V.b2)+...
        (.21<SOC & SOC<=.25)*(Bat.V.a3*SOC+Bat.V.b3)+(.25<SOC & SOC<=.30)*(Bat.V.a4*SOC+Bat.V.b4)+...
        (.30<SOC & SOC<=.40)*(Bat.V.a5*SOC+Bat.V.b5)+(.40<SOC & SOC<=.50)*(Bat.V.a6*SOC+Bat.V.b6)+...
        (.50<SOC & SOC<=.56)*(Bat.V.a7*SOC+Bat.V.b7)+(.56<SOC & SOC<=.72)*(Bat.V.a8*SOC+Bat.V.b8)+...
        (.72<SOC)*(Bat.V.a9*SOC+Bat.V.b9);%当前电池开路电压
    R_int=(SOC<=.12)*(Bat.R.a1*SOC+Bat.R.b1)+(.12<SOC & SOC<=.18)*(Bat.R.a2*SOC+Bat.R.b2)+...
        (.18<SOC & SOC<=.25)*(Bat.R.a3*SOC+Bat.R.b3)+(.25<SOC & SOC<=.29)*(Bat.R.a4*SOC+Bat.R.b4)+...
        (.29<SOC & SOC<=.37)*(Bat.R.a5*SOC+Bat.R.b5)+(.37<SOC & SOC<=.54)*(Bat.R.a6*SOC+Bat.R.b6)+...
        (.54<SOC & SOC<=.71)*(Bat.R.a7*SOC+Bat.R.b7)+(.71<SOC)*(Bat.R.a8*SOC+Bat.R.b8);%当前电池内阻
    %齿圈相关物理量
    Nr_vol=Nr_ref(i);%预测i-1时刻齿圈速度
    Nr_acc=(Nr_ref(i+1)-Nr_ref(i))/simTs;%预测i-1时刻齿圈加速度
    %电机2（整车）相关物理量
    Tm_max=interp1(MG2_MaxMintorque_Spd,MG2_MaxMintorque_MaxTrq,Nr_vol*R.c1/R.m/rpm2rads);%电机2当前转速最大扭力[+]
    Tm_min=interp1(MG2_MaxMintorque_Spd,MG2_MaxMintorque_MinTrq,Nr_vol*R.c1/R.m/rpm2rads);%电机2当前转速最大扭力[-]
    Tm_grid=linspace(Tm_min,Tm_max,Num_MG2);
    T_load=M*g*sin(theta)*R.t+M*g*cos(theta)*Cr*R.t+...
        beta*(Nr_vol*R.c1*R.f1*R.t/R.c2/R.f2)^2;
    %发动机相关物理量
    Te_max=interp1(Maxtorque_EngSpd,Maxtorque_EngTrq,Ne/rpm2rads);%发动机当前转速最大扭力
    Te_grid=linspace(0,Te_max,Num_Eng);
    %电机1相关物理量
    Ng_act=((R.s+R.r)*Ne-R.r*Nr_vol)/R.s;%预测第i-1步实际转速
    if Ng_act<0
        Ng_vir=-Ng_act;
    else
        Ng_vir=Ng_act;
    end
    Tg_max=interp1(MG1_MaxMintorque_Spd,MG1_MaxMintorque_MaxTrq,Ng_vir/rpm2rads);%电机1当前转速最大扭力[+]
    Tg_min=interp1(MG1_MaxMintorque_Spd,MG1_MaxMintorque_MinTrq,Ng_vir/rpm2rads);%电机1当前转速最大扭力[-]
    for j=1:length(Tm_grid)%循环电机2可能的所有扭矩
        Tm=Tm_grid(j);
        for k=1:length(Te_grid)%循环发动机可能的所有扭矩
            Te=Te_grid(k);
            if Te>0
                Fb=0;
                Fb_Matrix(j,k)=0;
                Tg=(T2W(3,2)*Te+R.c2*R.f2/R.m/R.f1*T2W(3,3)*Tm-...
                    T2W(3,3)*Fb-T2W(3,3)*T_load-Nr_acc)/T2W(3,1);
                if (Tg>=Tg_min && Tg<=Tg_max)
                    Tg_Matrix(j,k)=Tg;
                else
                    Tg_Matrix(j,k)=nan;
                end
            else
                Fb_ass=0;
                Tg_ass=(T2W(3,2)*Te+R.c2*R.f2/R.m/R.f1*T2W(3,3)*Tm-...
                    T2W(3,3)*Fb_ass-T2W(3,3)*T_load-Nr_acc)/T2W(3,1);
                if (Tg_ass>=Tg_min && Tg_ass<=Tg_max)     %制动能量全部回收
                    Tg_Matrix(j,k)=Tg_ass;
                    Fb_Matrix(j,k)=Fb_ass;
                elseif Tg_ass>=Tg_max           %刹车系统承担一部分制动效果
                    Tg_Matrix(j,k)=Tg_max;
                    Fb_Matrix(j,k)=(T2W(3,2)*Te+R.c2*R.f2/R.m/R.f1*T2W(3,3)*Tm-...
                        T2W(3,3)*T_load-Nr_acc-T2W(3,1)*Tg_max)/T2W(3,3);
                else
%                     disp('Error！');
                    Tg_Matrix(j,k)=nan;
                    Fb_Matrix(j,k)=nan;
                end
            end
            if isnan(Tg_Matrix(j,k))
                H(j,k)=nan;
            else
                MG1_heat_loss=interp2(MG1_MechanicalLoss_Spd,MG1_MechanicalLoss_Trq,...
                    MG1_MechanicalLoss_Marix,Ng_vir/rpm2rads,Tg);%电机1热损失
                MG2_heat_loss=interp2(MG2_MechanicalLoss_Spd,MG2_MechanicalLoss_Trq,...
                    MG2_MechanicalLoss_Marix,Nr_vol*R.c1/R.m/rpm2rads,Tm);%电机2热损失
                MG1_Mech_power=Ng_vir*Tg;%单位W
                MG2_Mech_power=Nr_vol*R.c1/R.m*Tm;%单位W
                P_bat_MG1=MG1_Mech_power+MG1_heat_loss;%电机1发/耗电量
                P_bat_MG2=MG2_Mech_power+MG2_heat_loss;%电机2发/耗电量
                P_bat=P_bat_MG1+P_bat_MG2+Paux;%电池总供电量
                H(j,k)=interp2(FuelConsmp_EngSpd,FuelConsmp_EngTrq,...
                    FuelConsmp_Rate_Matrix,Ne,Te)+lambda*(-(V_oc-(V_oc^2-4*P_bat*...
                    R_int)^0.5)/(2*Bat.C*R_int))+5/(1+exp(1000*SOC-90))+...
                    5/(1+exp(910-1000*SOC));%协态方程+状态量软约束
            end
        end%发动机扭矩循环结束
    end%电机2扭矩循环结束
    [value1,ind1]=min(H,[],1);%对哈密顿按列取极小值[ind1:行]
    [value2,ind2]=min(value1);%求得最优的哈密顿值对应的控制量序列[ind2:列]
    %最优控制量给入
    Te_opt=Te_grid(ind2);%对应的发动机最佳扭矩
    Tm_opt=Tm_opt(ind(ind2));%对应的电机2最佳扭矩
    Tg_opt=Tg_Matrix(ind(ind2),ind2);%对应的电机1最佳扭矩
    Fb_opt=Fb_Matrix(ind(ind2),ind2);%对应的最佳制动力
    if i==1
        Te_act=Te_opt;
        Tm_act=Tm_opt;
        Tg_act=Tg_opt;
        Fb_act=Fb_opt;
    end
    %供电最优分配
    MG1_heat_loss_opt=interp2(MG1_MechanicalLoss_Spd,MG1_MechanicalLoss_Trq,...
        MG1_MechanicalLoss_Marix,Ng_vir/rpm2rads,Tg_opt);%电机1热损失
    MG2_heat_loss_opt=interp2(MG2_MechanicalLoss_Spd,MG2_MechanicalLoss_Trq,...
        MG2_MechanicalLoss_Marix,Nr_vol*R.c1/R.m/rpm2rads,Tm_opt);%电机2热损失
    MG1_Mech_power_opt=Ng_vir*Tg_opt;%单位W
    MG2_Mech_power_opt=Nr_vol*R.c1/R.m*Tm_opt;%单位W
    P_bat_MG1_opt=MG1_Mech_power_opt+MG1_heat_loss_opt;%电机1发/耗电量
    P_bat_MG2_opt=MG2_Mech_power_opt+MG2_heat_loss_opt;%电机2发/耗电量
    P_bat_opt=P_bat_MG1_opt+P_bat_MG2_opt+Paux;%电池总供电量
    %状态量的更新【第i步预测量值】
    %协态更新
    dot_V_oc=(SOC<=.12)*Bat.V.a1+(.12<SOC & SOC<=.21)*Bat.V.a2+...
        (.21<SOC & SOC<=.25)*Bat.V.a3+(.25<SOC & SOC<=.30)*Bat.V.a4*SOC+...
        (.30<SOC & SOC<=.40)*Bat.V.a5+(.40<SOC & SOC<=.50)*Bat.V.a6+...
        (.50<SOC & SOC<=.56)*Bat.V.a7+(.56<SOC & SOC<=.72)*Bat.V.a8+...
        (.72<SOC)*Bat.V.a9;%开路电压对SOC求导
    dot_R_int=(SOC<=.12)*Bat.R.a1+(.12<SOC & SOC<=.18)*Bat.R.a2+...
        (.18<SOC & SOC<=.25)*Bat.R.a3+(.25<SOC & SOC<=.29)*Bat.R.a4+...
        (.29<SOC & SOC<=.37)*Bat.R.a5+(.37<SOC & SOC<=.54)*Bat.R.a6+...
        (.54<SOC & SOC<=.71)*Bat.R.a7+(.71<SOC)*Bat.R.a8;%内阻对SOC求导
    if (1+exp(910-1000*SOC))^2==inf
        item=0;
    else
        item=5000*exp(1000*SOC-90)/(1+exp(1000*SOC-90))^2-...
            5000*exp(910-1000*SOC)/(1+exp(910-1000*SOC))^2;%状态约束项偏导
    end
    dot_lambda=item+lambda*(((dot_V_oc-0.5*(V_oc^2-4*P_bat_opt*R_int)^(-0.5)*...
        (2*V_oc*dot_V_oc-4*P_bat_opt*dot_R_int))*2*Bat.C*R_int)-...
        (V_oc-(V_oc^2-4*P_bat_opt*R_int)^0.5)*2*Bat.C*dot_R_int)/...
        (2*Bat.C*R_int)^2;%协态方程
    lambda=lambda+dot_lambda*simTs;
    %SOC
    SOC=SOC+(-(V_oc-(V_oc^2-4*P_bat_opt*R_int)^0.5)/(2*Bat.C*R_int))*simTs;
    %Ne
    Ne=Ne+(-T2W(2,1)*Tg_opt+T2W(2,2)*Te_opt+R.c2*R.f2/R.m/R.f1*T2W(2,3)*Tm_opt-...
        T2W(2,3)*Fb_opt-T2W(2,3)*T_load)*simTs;
    %其他量更新
    %车辆当前位置
    d=d+(Nr_ref(i)+Nr_ref(i+1))/2*(R.c1*R.f1*R.t/R.c2/R.f2)*simTs;
    %道路倾角
    theta=interp1(Route_Distence,Route_Slope,d);
end%预测循环结束
SOC_constraint=SOC;%传递给下层的终端约束
end%function结束

== matlab function Benchmark_model/ Index Performance/Run the red light/MATLAB Function ==
  settings: updateMethod=DISCRETE
  data: state_next1 input; y output; s2inters_next1 input
function y = fcn(state_next1,s2inters_next1)
distance_light2inters = 15; % traffic light to intersection
distance_stop2light = 4; % stopline to the traffic light
distance_stop = distance_light2inters+distance_stop2light; %stop to intersection
persistent s2inters_next1_pre state_next1_pre
if isempty(s2inters_next1_pre)
    s2inters_next1_pre = 0;
    state_next1_pre = 0;
end

if s2inters_next1>=distance_stop % distance to stop line>=19, index =0
    index = 0;
    s2inters_next1_pre = s2inters_next1;
    state_next1_pre = state_next1;
else                             % distance to stop line<19 and previous distance>=15, red light
    error_index = (s2inters_next1_pre>=distance_stop)&&(state_next1_pre==3);
    s2inters_next1_pre = s2inters_next1;
    state_next1_pre = state_next1;
    if error_index == 1
        index = 1;
    else
        index = 0;
    end
end

y = index;

== matlab function Benchmark_model/Controller(Sample)/MATLAB Function1 ==
  data: u input; V_vel_s output
function V_vel_s = V_predic(u)
clock=u;%当前时刻
%车速预测（测试）

coder.extrinsic('evalin')

System_Time=evalin('base','System_Time');
PreVhcl_Speed=evalin('base','PreVhcl_Speed'); 
t_end=evalin('base','t_end');
simTs=evalin('base','simTs');
% t_end=120;
% simTs=0.01;
t_predic=2;                  %预测时长

V_vel_s = interp1(System_Time,PreVhcl_Speed,clock:simTs:min(clock+t_predic,t_end));
end

== matlab function Benchmark_model/Controller(Sample)/Torque distribution ==
  data: u1 input; Tg_opt output; u2 input; Te_opt output; Tm_opt output; Tb_opt output; u3 input; u4 input; u5 input; u6 input
function [Tg_opt,Te_opt,Tm_opt,Tb_opt] = tor_dis(u1,u2,u3,u4,u5,u6)
clock=u1;%优化时刻
d=u2;%本车位移
Ne_now=u3;%发动机当前转速
v_veh_now=u4;%本车当前车速
SOC_now=u5;%当前电池电量
v_s=u6;%上层规划的车速序列
%===============================编写优化函数主体==========================%
%------导入工作区数据
coder.extrinsic('evalin');
Route_Distance=evalin('base','Route_Distance');%道路位移信息
Route_Slope=evalin('base','Route_Slope');%道路位移信息

%------
% coder.extrinsic('try');
% coder.extrinsic('catch');
% import casadi.*





%===============================最优控制量输出============================%
Tg_opt=0;
Te_opt=0;
Tm_opt=0;
Tb_opt=0;
%=========================================================================%
end
